simulink model "task3_simulink"  (R2026a)
settings: Solver=VariableStepAuto  StopTime=2
settings Model: Creator=DELL  LastModifiedBy=DELL

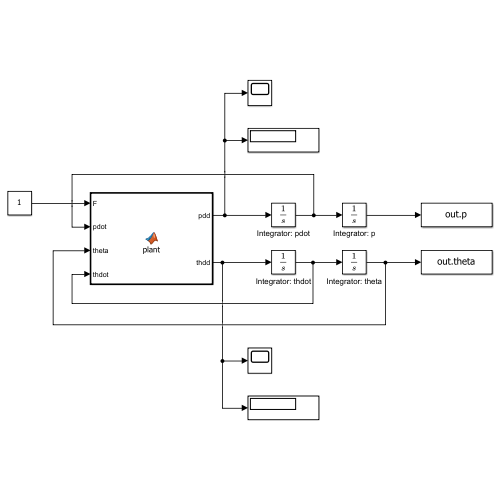
[thumbnail: Simulink's stored preview of the top-level diagram]
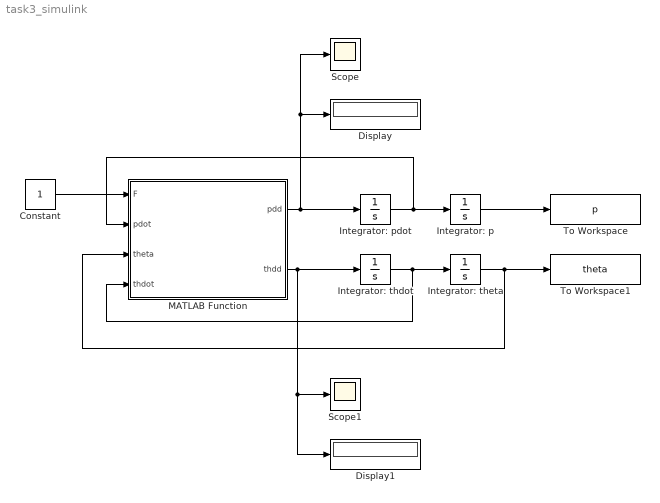
== system task3_simulink ==
  Constant : Constant
  Display : Display
  Display1 : Display
  Integrator: p : Integrator
  Integrator: pdot : Integrator
  Integrator: thdot : Integrator
  Integrator: theta : Integrator
  MATLAB Function : MATLAB Function  TreatAsAtomicUnit=on
  Scope : Scope
      settings: ActiveDisplayYMinimum=-0.39641230245518316  ActiveDisplayYMaximum=0.44251737136425118
  Scope1 : Scope
      settings: ActiveDisplayYMinimum=-17.991162422784569  ActiveDisplayYMaximum=13.047383471679943
  To Workspace : ToWorkspace  VariableName=p  SaveFormat=Timeseries  SampleTime=0.01
  To Workspace1 : ToWorkspace  VariableName=theta  SaveFormat=Timeseries  SampleTime=0.01
  wires:
  MATLAB Function/1(pdd) -> Display/1, Scope/1, Integrator: pdot/1
  MATLAB Function/2(thdd) -> Scope1/1, Display1/1, Integrator: thdot/1
  Integrator: pdot/1 -> MATLAB Function/2(pdot), Integrator: p/1
  Integrator: thdot/1 -> MATLAB Function/4(thdot), Integrator: theta/1
  Integrator: theta/1 -> To Workspace1/1, MATLAB Function/3(theta)
  Constant/1 -> MATLAB Function/1(F)
  Integrator: p/1 -> To Workspace/1

== matlab function task3_simulink/MATLAB Function ==
  data: F input; pdd output; pdot input; theta input; thdot input; thdd output
function [pdd, thdd] = plant(F, pdot, theta, thdot)

M = 5;
m = 1;
l = 0.5;
c = 0.2;
g = 9.8;

pdd = ( ...
    F ...
    - c*pdot ...
    + m*g*sin(theta)*cos(theta) ...
    - m*l*sin(theta)*thdot^2 ...
    ) / (M+m-m*cos(theta)^2);

thdd = ( ...
    cos(theta)*pdd ...
    + g*sin(theta) ...
    ) / l;

end
